simulink model "snap_adc5g_spec"  (R2019a)
settings: Solver=VariableStepDiscrete  StartTime=0.0  StopTime=10.0  RelTol=1e-3
undefined symbols (not defined in the file): pfb_coeff_gen_calc
libraries: xbsIndex_r4 x13965, casper_library_misc x80, casper_library_delays x43, xps_library x5, xbsReplacements_r4 x2, casper_library_communications x1
(part 127 of 152)

== system snap_adc5g_spec/fft_wideband_real/fft_biplex_real_4x/biplex_core/fft_stage_9/butterfly_direct/twiddle/bus_mult ==
  a : Inport
  b : Inport  Port=2
  misci : Inport  Port=3
  a*b_bussify : Subsystem  AncestorBlock=casper_library_flow_control/bus_create  mask(bus_create){inputNum=2}
      mask prompts: inputNum "Number of inputs:"
      mask init:
      | bus_create_init(gcb,...
      |     'inputNum', inputNum);
  a_debus : Subsystem  AncestorBlock=casper_library_flow_control/bus_expand  mask(bus_expand){mode=divisions of arbitrary size, outputNum=1, outputWidth=36, outputBinaryPt=0, outputArithmeticType=0, show_format=on, outputToWorkspace=off, variablePrefix=, outputToModelAsWell=on}
      mask prompts: outputNum "Number of outputs:"; outputWidth "Output width [msb ... lsb]:"; outputBinaryPt "Output binary point position [msb ... lsb]:"; outputArithmeticType "Output arithmetic type (ufix=0, fix=1, bool=2) [msb ... lsb]:"; show_format "Print format string?"; outputToWorkspace "Output to workspace?"; variablePrefix "Variable name prefix:"; outputToModelAsWell "Output to model as well?"
      mask help:
      | Expands a 'bus' made using a bus_create or Xilinx
      | concat block.
      | The input will be divided into the specified number
      | of outputs with the specified arithmetic types.
      | Divisions are made from most significant bit.
      mask init: same as snap_adc5g_spec/ss_adc/ctrl_split
      settings: AttributesFormatString=1 outputs: uf36.0,
      mask TypeOptions mode: divisions of equal size | divisions of arbitrary size
      mask Callback mode: bus_expand_callback();
      mask Callback outputWidth: bus_expand_callback();
      mask Callback outputToWorkspace: bus_expand_callback();
  b_debus : Subsystem  AncestorBlock=casper_library_flow_control/bus_expand  mask(bus_expand){mode=divisions of arbitrary size, outputNum=1, outputWidth=[36 36], outputBinaryPt=[0 0], outputArithmeticType=[0 0], show_format=on, outputToWorkspace=off, variablePrefix=, outputToModelAsWell=on}
      mask prompts: outputNum "Number of outputs:"; outputWidth "Output width [msb ... lsb]:"; outputBinaryPt "Output binary point position [msb ... lsb]:"; outputArithmeticType "Output arithmetic type (ufix=0, fix=1, bool=2) [msb ... lsb]:"; show_format "Print format string?"; outputToWorkspace "Output to workspace?"; variablePrefix "Variable name prefix:"; outputToModelAsWell "Output to model as well?"
      mask help:
      | Expands a 'bus' made using a bus_create or Xilinx
      | concat block.
      | The input will be divided into the specified number
      | of outputs with the specified arithmetic types.
      | Divisions are made from most significant bit.
      mask init: same as snap_adc5g_spec/ss_adc/ctrl_split
      settings: AttributesFormatString=2 outputs: uf36.0,uf36.0,
      mask TypeOptions mode: divisions of equal size | divisions of arbitrary size
      mask Callback mode: bus_expand_callback();
      mask Callback outputWidth: bus_expand_callback();
      mask Callback outputToWorkspace: bus_expand_callback();
  dmisc : xbsIndex_r4/Delay  rst=off  infoeditControl=Selection of Reset will increase slice count due to use of real FFs and instead of SRLs  en=off  latency=mult_latency+add_latency+conv_latency+fan_latency  reg_retiming=on  dbl_ovrd=off  block_type=delay
  mult1 : Subsystem  AncestorBlock=casper_library_multipliers/cmult  mask(cmult){n_bits_a=18, bin_pt_a=17, n_bits_b=18, bin_pt_b=17, n_bits_ab=37, bin_pt_ab=34, quantization=Truncate, overflow=Wrap, conjugated=off, async=off, pipelined_enable=on, floating_point=off, float_type=single, exp_width=8, frac_width=24, in_latency=1, mult_latency=2, add_latency=1, conv_latency=0, pipeline_cmult_en=off, pipeline_latency=0, multiplier_implementation=behavioral HDL}
      mask prompts: n_bits_a "Number of Bits 'a'"; bin_pt_a "Binary Point 'a'"; n_bits_b "Number of Bits 'b'"; bin_pt_b "Binary Point 'b'"; n_bits_ab "Number of Bits 'ab'"; bin_pt_ab "Binary Point 'ab'"; conjugated "Conjugate"; async "asynchronous operation"; pipelined_enable "enable pipeline"; floating_point "floating point"; float_type "float type"; exp_width "exponent width"; frac_width "fraction width"; in_latency "Input latency"; mult_latency "Multiplier Latency"; add_latency "Adder Latency"; conv_latency "Convert latency"; pipeline_cmult_en "Pipeline cmult enable"; pipeline_latency "Pipeline latency"; multiplier_implementation "Multiplier implementation"
      mask help:
      | Multiplies two complex numbers using 4 multipliers and 2 adders.
      | Conjugation is optional.
      mask init: same as snap_adc5g_spec/crosspower_vacc/cmult
      settings: AttributesFormatString=|
      | 18_17 * 18_17 ==> 37_34
      | Truncate, Wrap
      | Latency=1
      mask TypeOptions quantization: Truncate | Round  (unbiased: +/- Inf) | Round  (unbiased: Even Values)
      mask TypeOptions overflow: Wrap | Saturate | Flag as error
      mask Callback floating_point:
      | onoff = get_param(gcb, 'floating_point');
      | if strcmp(onoff,'on')
      |     enable_fixpt = 'off'
      |     set_param_state(gcb, 'float_type', 'on')
      | 
      |     f_type = get_param(gcb, 'float_type')
      |     if strcmp(f_type,'custom')
      |         set_param_state(gcb, 'exp_width', 'on')
      |         set_param_state(gcb, 'frac_width', 'on')
      |     else
      |         set_param_state(gcb, 'exp_width', 'off')
      |         set_param_state(gcb, 'frac_width', 'off')
      |     end
      | 
      | 
      | else
      |     enable_fixpt = 'on'
      |     set_param_state(gcb, 'float_type', 'off')
      |     set_param_state(gcb, 'exp_width', 'off')
      |     set_param_state(gcb, 'frac_width', 'off')
      | end
      | 
      | 
      | set_param_state(gcb, 'n_bits_a', enable_fixpt)
      | set_param_state(gcb, 'bin_pt_a', enable_fixpt)
      | set_param_state(gcb, 'n_bits_b', enable_fixpt)
      | set_param_state(gcb, 'bin_pt_b', enable_fixpt)
      | set_param_state(gcb, 'n_bits_ab', enable_fixpt)
      | set_param_state(gcb, 'bin_pt_ab', enable_fixpt)
      mask TypeOptions float_type: single | custom
      mask Callback float_type:
      | f_type = get_param(gcb, 'float_type')
      | if strcmp(f_type,'custom')
      |     set_param_state(gcb, 'exp_width', 'on')
      |     set_param_state(gcb, 'frac_width', 'on')
      | else
      |     set_param_state(gcb, 'exp_width', 'off')
      |     set_param_state(gcb, 'frac_width', 'off')
      | end
      mask Callback pipeline_cmult_en:
      | pipeline_en = get_param(gcb, 'pipeline_cmult_en');
      | if strcmp(pipeline_en,'on')
      | 
      |     set_param_state(gcb, 'pipeline_latency', 'on')
      | else
      |     set_param_state(gcb, 'pipeline_latency', 'off')
      | end
      mask TypeOptions multiplier_implementation: behavioral HDL | standard core | embedded multiplier core
      mask DialogControl ParameterTabVar0 Prompt: basic
      mask DialogControl ParameterTabVar01 Prompt: latency
      mask DialogControl ParameterTabVar012 Prompt: implementation
  mult2 : Subsystem  AncestorBlock=casper_library_multipliers/cmult  mask(cmult){n_bits_a=18, bin_pt_a=17, n_bits_b=18, bin_pt_b=17, n_bits_ab=37, bin_pt_ab=34, quantization=Truncate, overflow=Wrap, conjugated=off, async=off, pipelined_enable=on, floating_point=off, float_type=single, exp_width=8, frac_width=24, in_latency=1, mult_latency=2, add_latency=1, conv_latency=0, pipeline_cmult_en=off, pipeline_latency=0, multiplier_implementation=behavioral HDL}
      mask prompts: n_bits_a "Number of Bits 'a'"; bin_pt_a "Binary Point 'a'"; n_bits_b "Number of Bits 'b'"; bin_pt_b "Binary Point 'b'"; n_bits_ab "Number of Bits 'ab'"; bin_pt_ab "Binary Point 'ab'"; conjugated "Conjugate"; async "asynchronous operation"; pipelined_enable "enable pipeline"; floating_point "floating point"; float_type "float type"; exp_width "exponent width"; frac_width "fraction width"; in_latency "Input latency"; mult_latency "Multiplier Latency"; add_latency "Adder Latency"; conv_latency "Convert latency"; pipeline_cmult_en "Pipeline cmult enable"; pipeline_latency "Pipeline latency"; multiplier_implementation "Multiplier implementation"
      mask help:
      | Multiplies two complex numbers using 4 multipliers and 2 adders.
      | Conjugation is optional.
      mask init: same as snap_adc5g_spec/crosspower_vacc/cmult
      settings: AttributesFormatString=|
      | 18_17 * 18_17 ==> 37_34
      | Truncate, Wrap
      | Latency=1
      mask TypeOptions quantization: Truncate | Round  (unbiased: +/- Inf) | Round  (unbiased: Even Values)
      mask TypeOptions overflow: Wrap | Saturate | Flag as error
      mask Callback floating_point:
      | onoff = get_param(gcb, 'floating_point');
      | if strcmp(onoff,'on')
      |     enable_fixpt = 'off'
      |     set_param_state(gcb, 'float_type', 'on')
      | 
      |     f_type = get_param(gcb, 'float_type')
      |     if strcmp(f_type,'custom')
      |         set_param_state(gcb, 'exp_width', 'on')
      |         set_param_state(gcb, 'frac_width', 'on')
      |     else
      |         set_param_state(gcb, 'exp_width', 'off')
      |         set_param_state(gcb, 'frac_width', 'off')
      |     end
      | 
      | 
      | else
      |     enable_fixpt = 'on'
      |     set_param_state(gcb, 'float_type', 'off')
      |     set_param_state(gcb, 'exp_width', 'off')
      |     set_param_state(gcb, 'frac_width', 'off')
      | end
      | 
      | 
      | set_param_state(gcb, 'n_bits_a', enable_fixpt)
      | set_param_state(gcb, 'bin_pt_a', enable_fixpt)
      | set_param_state(gcb, 'n_bits_b', enable_fixpt)
      | set_param_state(gcb, 'bin_pt_b', enable_fixpt)
      | set_param_state(gcb, 'n_bits_ab', enable_fixpt)
      | set_param_state(gcb, 'bin_pt_ab', enable_fixpt)
      mask TypeOptions float_type: single | custom
      mask Callback float_type:
      | f_type = get_param(gcb, 'float_type')
      | if strcmp(f_type,'custom')
      |     set_param_state(gcb, 'exp_width', 'on')
      |     set_param_state(gcb, 'frac_width', 'on')
      | else
      |     set_param_state(gcb, 'exp_width', 'off')
      |     set_param_state(gcb, 'frac_width', 'off')
      | end
      mask Callback pipeline_cmult_en:
      | pipeline_en = get_param(gcb, 'pipeline_cmult_en');
      | if strcmp(pipeline_en,'on')
      | 
      |     set_param_state(gcb, 'pipeline_latency', 'on')
      | else
      |     set_param_state(gcb, 'pipeline_latency', 'off')
      | end
      mask TypeOptions multiplier_implementation: behavioral HDL | standard core | embedded multiplier core
      mask DialogControl ParameterTabVar0 Prompt: basic
      mask DialogControl ParameterTabVar01 Prompt: latency
      mask DialogControl ParameterTabVar012 Prompt: implementation
  repa : Subsystem  AncestorBlock=casper_library_bus/bus_replicate  mask(bus_replicate){replication=1, csp_latency=1, misc=off, implementation=core}
      mask prompts: replication "replication factor"; csp_latency "latency"; misc "misc support"; implementation "delay implementation"
      mask help: Output bus formed by replicating input bus a number of times
      mask init:
      | bus_replicate_init(gcb, ...
      |     'replication', replication, ...
      |     'csp_latency', csp_latency, ...
      |     'implementation', implementation, ...
      |     'misc', misc);
      mask TypeOptions implementation: core | behavioral
  repb : Subsystem  AncestorBlock=casper_library_bus/bus_replicate  mask(bus_replicate){replication=1, csp_latency=1, misc=off, implementation=core}
      mask prompts: replication "replication factor"; csp_latency "latency"; misc "misc support"; implementation "delay implementation"
      mask help: Output bus formed by replicating input bus a number of times
      mask init:
      | bus_replicate_init(gcb, ...
      |     'replication', replication, ...
      |     'csp_latency', csp_latency, ...
      |     'implementation', implementation, ...
      |     'misc', misc);
      mask TypeOptions implementation: core | behavioral
  a*b : Outport
  misco : Outport  Port=2
  wires:
  a/1 -> repa/1(in)
  b/1 -> repb/1(in)
  repa/1(out) -> a_debus/1(bus_in)
  repb/1(out) -> b_debus/1(bus_in)
  a_debus/1(msb_lsb_out1) -> mult1/1(a), mult2/1(a)
  b_debus/1(msb_out2) -> mult1/2(b)
  b_debus/2(lsb_out1) -> mult2/2(b)
  misci/1 -> dmisc/1
  mult1/1(ab) -> a*b_bussify/1(in1)
  mult2/1(ab) -> a*b_bussify/2(in2)
  a*b_bussify/1(bus_out) -> a*b/1
  dmisc/1 -> misco/1

== system snap_adc5g_spec/fft_wideband_real/fft_biplex_real_4x/biplex_core/fft_stage_9/butterfly_direct/twiddle/coeff_gen ==
  rst : Inport
  misci : Inport  Port=2
  Counter : xbsIndex_r4/Counter  cnt_type=Free Running  cnt_to=Inf  operation=Up  start_count=0  cnt_by_val=1  arith_type=Unsigned  n_bits=10  bin_pt=0  load_pin=off  rst=on  en=off  explicit_period=on  period=1  use_behavioral_HDL=on  implementation=Fabric  dbl_ovrd=off  block_type=counter
  Slice : xbsIndex_r4/Slice  nbits=8  boolean_output=off  mode=Upper Bit Location + Width  bit1=0  base1=MSB of Input  bit0=0  base0=LSB of Input  dbl_ovrd=off  block_type=slice
  bit_reverse : Subsystem  AncestorBlock=casper_library_misc/bit_reverse  mask(bit_reverse){n_bits=8}
      mask prompts: n_bits "Number of Bits"
      mask help: Reverses the bit order of the input. Input must be unsigned with binary point at position 0. Costs nothing in hardware.
      mask init:
      | bit_reverse_init(gcb,'n_bits', n_bits);
      settings: AttributesFormatString=8 bits
      mask Help: eval('xlWeb(''http://casper.berkeley.edu/wiki/Bit_reverse'')')
  cosin : Subsystem  Tag=casper:cosin  AncestorBlock=casper_library_downconverter/cosin  mask(cosin){output0=cos, output1=-sin, indep_theta=off, phase=0, fraction=1, table_bits=8, n_bits=18, bin_pt=17, floating_point=off, float_type=single, exp_width=8, frac_width=24, store=1, pack=on, bram=BRAM, misc=on, bram_latency=3, add_latency=1, mux_latency=2, neg_latency=2, conv_latency=1}
      mask prompts: output0 "first output function"; output1 "second output function"; indep_theta "Independent theta values"; phase "initial phase offset (?*(2*pi))"; fraction "fraction of cycle period to output (1/2^?)"; table_bits "samples in cycle period fraction to output (2^?)"; n_bits "bit width"; bin_pt "binary point"; floating_point "floating point"; float_type "float type"; exp_width "exponent width"; frac_width "fraction width"; store "fraction of cycle period to store (1/2^?)"; pack "pack lookup values in same output word"; bram "BRAM implementation"; misc "Miscellaneous port"; bram_latency "bram latency"; add_latency "large adder latency"; mux_latency "mux latency"; neg_latency "negate latency"; conv_latency "convert latency"
      mask init: same as snap_adc5g_spec/fft_wideband_real/fft_direct/butterfly0_0/twiddle/coeff_gen/cosin
      mask TypeOptions output0: sin | cos | -sin | -cos
      mask TypeOptions output1: none | sin | cos | -sin | -cos
      mask Callback floating_point:
      | onoff = get_param(gcb, 'floating_point');
      | if strcmp(onoff,'on')
      |     enable_fixpt = 'off';
      |     set_param_state(gcb, 'float_type', 'on')
      | 
      |     f_type = get_param(gcb, 'float_type');
      |     if strcmp(f_type,'custom')
      |         set_param_state(gcb, 'exp_width', 'on')
      |         set_param_state(gcb, 'frac_width', 'on')
      |     else
      |         set_param_state(gcb, 'exp_width', 'off')
      |         set_param_state(gcb, 'frac_width', 'off')
      |     end
      | 
      | 
      | else
      |     enable_fixpt = 'on';
      |     set_param_state(gcb, 'float_type', 'off')
      |     set_param_state(gcb, 'exp_width', 'off')
      |     set_param_state(gcb, 'frac_width', 'off')
      | end
      | 
      | set_param_state(gcb, 'n_bits', enable_fixpt)
      | set_param_state(gcb, 'bin_pt', enable_fixpt)
      mask TypeOptions float_type: single | custom
      mask Callback float_type:
      | f_type = get_param(gcb, 'float_type');
      | if strcmp(f_type,'custom')
      |     set_param_state(gcb, 'exp_width', 'on')
      |     set_param_state(gcb, 'frac_width', 'on')
      | else
      |     set_param_state(gcb, 'exp_width', 'off')
      |     set_param_state(gcb, 'frac_width', 'off')
      | end
      mask TypeOptions bram: distributed RAM | BRAM
      mask Display:
      | if ~(table_bits == 0),
      |         color('black');port_label('output',1,output0);
      |     color('black');port_label('output',2,output1);
      |     color('black');disp(['z^{-',num2str(add_latency+mux_latency+conv_latency+bram_latency+neg_latency+mux_latency),'}'],'texmode','on');color('black');port_label('input',1,'theta');
      |     if strcmp(misc, 'on'),
      |         color('black');port_label('input',2,'misci');
      |         color('black');port_label('output',3,'misco');
      |     end
      | end
  ri_to_c : casper_library_misc/ri_to_c
      settings: SourceProductName=CASPER DSP Blockset
  w : Outport
  misco : Outport  Port=2
  wires:
  ri_to_c/1 -> w/1
  rst/1 -> Counter/1
  Counter/1 -> Slice/1
  Slice/1 -> bit_reverse/1(in)
  bit_reverse/1(out) -> cosin/1(theta)
  cosin/1(cos) -> ri_to_c/1
  cosin/2(-sin) -> ri_to_c/2
  misci/1 -> cosin/2(misci)
  cosin/3(misco) -> misco/1

== system snap_adc5g_spec/fft_wideband_real/fft_direct/butterfly0_0/twiddle/bus_mult/mult1/a_expand ==
  bus_in : Inport
  reinterpret{1..4} (4 alike) : xbsIndex_r4/Reinterpret  force_arith_type=on  arith_type="Signed  (2's comp)"  force_bin_pt=on  bin_pt=17  block_type=reinterpret
  slice1 : xbsIndex_r4/Slice  nbits=18  boolean_output=off  mode=Upper Bit Location + Width  bit1=-54  base1=MSB of Input  bit0=0  base0=LSB of Input  dbl_ovrd=off  block_type=slice
  slice2 : xbsIndex_r4/Slice  nbits=18  boolean_output=off  mode=Upper Bit Location + Width  bit1=-36  base1=MSB of Input  bit0=0  base0=LSB of Input  dbl_ovrd=off  block_type=slice
  slice3 : xbsIndex_r4/Slice  nbits=18  boolean_output=off  mode=Upper Bit Location + Width  bit1=-18  base1=MSB of Input  bit0=0  base0=LSB of Input  dbl_ovrd=off  block_type=slice
  slice4 : xbsIndex_r4/Slice  nbits=18  boolean_output=off  mode=Upper Bit Location + Width  bit1=0  base1=MSB of Input  bit0=0  base0=LSB of Input  dbl_ovrd=off  block_type=slice
  msb_out4 : Outport
  out3 : Outport  Port=2
  out2 : Outport  Port=3
  lsb_out1 : Outport  Port=4
  wires:
  bus_in/1 -> slice4/1, slice3/1, slice2/1, slice1/1
  slice4/1 -> reinterpret4/1
  reinterpret4/1 -> msb_out4/1
  slice3/1 -> reinterpret3/1
  reinterpret3/1 -> out3/1
  slice2/1 -> reinterpret2/1
  reinterpret2/1 -> out2/1
  slice1/1 -> reinterpret1/1
  reinterpret1/1 -> lsb_out1/1

== system snap_adc5g_spec/fft_wideband_real/fft_direct/butterfly0_0/twiddle/bus_mult/mult1/a_replicate ==
  in : Inport
  bussify : Subsystem  AncestorBlock=casper_library_flow_control/bus_create  mask(bus_create){inputNum=2}
      mask prompts: inputNum "Number of inputs:"
      mask init:
      | bus_create_init(gcb,...
      |     'inputNum', inputNum);
  din0_0 : xbsIndex_r4/Delay  rst=off  infoeditControl=Selection of Reset will increase slice count due to use of real FFs and instead of SRLs  en=off  latency=1  reg_retiming=off  dbl_ovrd=off  block_type=delay
  din0_1 : xbsIndex_r4/Delay  rst=off  infoeditControl=Selection of Reset will increase slice count due to use of real FFs and instead of SRLs  en=off  latency=1  reg_retiming=off  dbl_ovrd=off  block_type=delay
  out : Outport
  wires:
  in/1 -> din0_0/1, din0_1/1
  din0_0/1 -> bussify/1(in1)
  din0_1/1 -> bussify/2(in2)
  bussify/1(bus_out) -> out/1

== system snap_adc5g_spec/fft_wideband_real/fft_direct/butterfly0_0/twiddle/bus_mult/mult1/b_expand ==
  bus_in : Inport
  reinterpret{1..4} (4 alike) : xbsIndex_r4/Reinterpret  force_arith_type=on  arith_type="Signed  (2's comp)"  force_bin_pt=on  bin_pt=17  block_type=reinterpret
  slice1 : xbsIndex_r4/Slice  nbits=18  boolean_output=off  mode=Upper Bit Location + Width  bit1=-54  base1=MSB of Input  bit0=0  base0=LSB of Input  dbl_ovrd=off  block_type=slice
  slice2 : xbsIndex_r4/Slice  nbits=18  boolean_output=off  mode=Upper Bit Location + Width  bit1=-36  base1=MSB of Input  bit0=0  base0=LSB of Input  dbl_ovrd=off  block_type=slice
  slice3 : xbsIndex_r4/Slice  nbits=18  boolean_output=off  mode=Upper Bit Location + Width  bit1=-18  base1=MSB of Input  bit0=0  base0=LSB of Input  dbl_ovrd=off  block_type=slice
  slice4 : xbsIndex_r4/Slice  nbits=18  boolean_output=off  mode=Upper Bit Location + Width  bit1=0  base1=MSB of Input  bit0=0  base0=LSB of Input  dbl_ovrd=off  block_type=slice
  msb_out4 : Outport
  out3 : Outport  Port=2
  out2 : Outport  Port=3
  lsb_out1 : Outport  Port=4
  wires:
  bus_in/1 -> slice4/1, slice3/1, slice2/1, slice1/1
  slice4/1 -> reinterpret4/1
  reinterpret4/1 -> msb_out4/1
  slice3/1 -> reinterpret3/1
  reinterpret3/1 -> out3/1
  slice2/1 -> reinterpret2/1
  reinterpret2/1 -> out2/1
  slice1/1 -> reinterpret1/1
  reinterpret1/1 -> lsb_out1/1

== system snap_adc5g_spec/fft_wideband_real/fft_direct/butterfly0_0/twiddle/bus_mult/mult1/b_replicate ==
  in : Inport
  bussify : Subsystem  AncestorBlock=casper_library_flow_control/bus_create  mask(bus_create){inputNum=2}
      mask prompts: inputNum "Number of inputs:"
      mask init:
      | bus_create_init(gcb,...
      |     'inputNum', inputNum);
  din0_0 : xbsIndex_r4/Delay  rst=off  infoeditControl=Selection of Reset will increase slice count due to use of real FFs and instead of SRLs  en=off  latency=1  reg_retiming=off  dbl_ovrd=off  block_type=delay
  din0_1 : xbsIndex_r4/Delay  rst=off  infoeditControl=Selection of Reset will increase slice count due to use of real FFs and instead of SRLs  en=off  latency=1  reg_retiming=off  dbl_ovrd=off  block_type=delay
  out : Outport
  wires:
  in/1 -> din0_0/1, din0_1/1
  din0_0/1 -> bussify/1(in1)
  din0_1/1 -> bussify/2(in2)
  bussify/1(bus_out) -> out/1

== system snap_adc5g_spec/fft_wideband_real/fft_direct/butterfly0_0/twiddle/bus_mult/mult1/ri_to_c ==
  re : Inport
  im : Inport  Port=2
  concat : xbsIndex_r4/Concat  num_inputs=2  dbl_ovrd=off  block_type=concat
      settings: block_version=9.1.01
  force_im : xbsIndex_r4/Reinterpret  force_arith_type=on  arith_type=Unsigned  force_bin_pt=on  bin_pt=0  block_type=reinterpret
      settings: infoedit="Changes signal type without altering the binary representation.   You can changed the signal between signed and unsigned, and relocate the binary point.<P><P>Hardware notes: In hardware this block costs nothing.<P><P>Example:  Suppose the input is 6 bits wide, signed, with 2 fractional bits, and the output is forced to unsigned with 0 fractional bits.  Then an input of -2.0 (1110.00 in binary 2's complement) becomes an output of 56 (111000 in binary)."  block_version=9.1.01
  force_re : xbsIndex_r4/Reinterpret  force_arith_type=on  arith_type=Unsigned  force_bin_pt=on  bin_pt=0  block_type=reinterpret
      settings: infoedit="Changes signal type without altering the binary representation.   You can changed the signal between signed and unsigned, and relocate the binary point.<P><P>Hardware notes: In hardware this block costs nothing.<P><P>Example:  Suppose the input is 6 bits wide, signed, with 2 fractional bits, and the output is forced to unsigned with 0 fractional bits.  Then an input of -2.0 (1110.00 in binary 2's complement) becomes an output of 56 (111000 in binary)."  block_version=9.1.01
  c : Outport
  wires:
  force_re/1 -> concat/1
  force_im/1 -> concat/2
  re/1 -> force_re/1
  concat/1 -> c/1
  im/1 -> force_im/1

== system snap_adc5g_spec/fft_wideband_real/fft_direct/butterfly0_0/twiddle/bus_mult/mult2/a_expand ==
  bus_in : Inport
  reinterpret{1..4} (4 alike) : xbsIndex_r4/Reinterpret  force_arith_type=on  arith_type="Signed  (2's comp)"  force_bin_pt=on  bin_pt=17  block_type=reinterpret
  slice1 : xbsIndex_r4/Slice  nbits=18  boolean_output=off  mode=Upper Bit Location + Width  bit1=-54  base1=MSB of Input  bit0=0  base0=LSB of Input  dbl_ovrd=off  block_type=slice
  slice2 : xbsIndex_r4/Slice  nbits=18  boolean_output=off  mode=Upper Bit Location + Width  bit1=-36  base1=MSB of Input  bit0=0  base0=LSB of Input  dbl_ovrd=off  block_type=slice
  slice3 : xbsIndex_r4/Slice  nbits=18  boolean_output=off  mode=Upper Bit Location + Width  bit1=-18  base1=MSB of Input  bit0=0  base0=LSB of Input  dbl_ovrd=off  block_type=slice
  slice4 : xbsIndex_r4/Slice  nbits=18  boolean_output=off  mode=Upper Bit Location + Width  bit1=0  base1=MSB of Input  bit0=0  base0=LSB of Input  dbl_ovrd=off  block_type=slice
  msb_out4 : Outport
  out3 : Outport  Port=2
  out2 : Outport  Port=3
  lsb_out1 : Outport  Port=4
  wires:
  bus_in/1 -> slice4/1, slice3/1, slice2/1, slice1/1
  slice4/1 -> reinterpret4/1
  reinterpret4/1 -> msb_out4/1
  slice3/1 -> reinterpret3/1
  reinterpret3/1 -> out3/1
  slice2/1 -> reinterpret2/1
  reinterpret2/1 -> out2/1
  slice1/1 -> reinterpret1/1
  reinterpret1/1 -> lsb_out1/1

== system snap_adc5g_spec/fft_wideband_real/fft_direct/butterfly0_0/twiddle/bus_mult/mult2/a_replicate ==
  in : Inport
  bussify : Subsystem  AncestorBlock=casper_library_flow_control/bus_create  mask(bus_create){inputNum=2}
      mask prompts: inputNum "Number of inputs:"
      mask init:
      | bus_create_init(gcb,...
      |     'inputNum', inputNum);
  din0_0 : xbsIndex_r4/Delay  rst=off  infoeditControl=Selection of Reset will increase slice count due to use of real FFs and instead of SRLs  en=off  latency=1  reg_retiming=off  dbl_ovrd=off  block_type=delay
  din0_1 : xbsIndex_r4/Delay  rst=off  infoeditControl=Selection of Reset will increase slice count due to use of real FFs and instead of SRLs  en=off  latency=1  reg_retiming=off  dbl_ovrd=off  block_type=delay
  out : Outport
  wires:
  in/1 -> din0_0/1, din0_1/1
  din0_0/1 -> bussify/1(in1)
  din0_1/1 -> bussify/2(in2)
  bussify/1(bus_out) -> out/1

== system snap_adc5g_spec/fft_wideband_real/fft_direct/butterfly0_0/twiddle/bus_mult/mult2/b_expand ==
  bus_in : Inport
  reinterpret{1..4} (4 alike) : xbsIndex_r4/Reinterpret  force_arith_type=on  arith_type="Signed  (2's comp)"  force_bin_pt=on  bin_pt=17  block_type=reinterpret
  slice1 : xbsIndex_r4/Slice  nbits=18  boolean_output=off  mode=Upper Bit Location + Width  bit1=-54  base1=MSB of Input  bit0=0  base0=LSB of Input  dbl_ovrd=off  block_type=slice
  slice2 : xbsIndex_r4/Slice  nbits=18  boolean_output=off  mode=Upper Bit Location + Width  bit1=-36  base1=MSB of Input  bit0=0  base0=LSB of Input  dbl_ovrd=off  block_type=slice
  slice3 : xbsIndex_r4/Slice  nbits=18  boolean_output=off  mode=Upper Bit Location + Width  bit1=-18  base1=MSB of Input  bit0=0  base0=LSB of Input  dbl_ovrd=off  block_type=slice
  slice4 : xbsIndex_r4/Slice  nbits=18  boolean_output=off  mode=Upper Bit Location + Width  bit1=0  base1=MSB of Input  bit0=0  base0=LSB of Input  dbl_ovrd=off  block_type=slice
  msb_out4 : Outport
  out3 : Outport  Port=2
  out2 : Outport  Port=3
  lsb_out1 : Outport  Port=4
  wires:
  bus_in/1 -> slice4/1, slice3/1, slice2/1, slice1/1
  slice4/1 -> reinterpret4/1
  reinterpret4/1 -> msb_out4/1
  slice3/1 -> reinterpret3/1
  reinterpret3/1 -> out3/1
  slice2/1 -> reinterpret2/1
  reinterpret2/1 -> out2/1
  slice1/1 -> reinterpret1/1
  reinterpret1/1 -> lsb_out1/1

== system snap_adc5g_spec/fft_wideband_real/fft_direct/butterfly0_0/twiddle/bus_mult/mult2/b_replicate ==
  in : Inport
  bussify : Subsystem  AncestorBlock=casper_library_flow_control/bus_create  mask(bus_create){inputNum=2}
      mask prompts: inputNum "Number of inputs:"
      mask init:
      | bus_create_init(gcb,...
      |     'inputNum', inputNum);
  din0_0 : xbsIndex_r4/Delay  rst=off  infoeditControl=Selection of Reset will increase slice count due to use of real FFs and instead of SRLs  en=off  latency=1  reg_retiming=off  dbl_ovrd=off  block_type=delay
  din0_1 : xbsIndex_r4/Delay  rst=off  infoeditControl=Selection of Reset will increase slice count due to use of real FFs and instead of SRLs  en=off  latency=1  reg_retiming=off  dbl_ovrd=off  block_type=delay
  out : Outport
  wires:
  in/1 -> din0_0/1, din0_1/1
  din0_0/1 -> bussify/1(in1)
  din0_1/1 -> bussify/2(in2)
  bussify/1(bus_out) -> out/1

== system snap_adc5g_spec/fft_wideband_real/fft_direct/butterfly0_0/twiddle/bus_mult/mult2/ri_to_c ==
  re : Inport
  im : Inport  Port=2
  concat : xbsIndex_r4/Concat  num_inputs=2  dbl_ovrd=off  block_type=concat
      settings: block_version=9.1.01
  force_im : xbsIndex_r4/Reinterpret  force_arith_type=on  arith_type=Unsigned  force_bin_pt=on  bin_pt=0  block_type=reinterpret
      settings: infoedit="Changes signal type without altering the binary representation.   You can changed the signal between signed and unsigned, and relocate the binary point.<P><P>Hardware notes: In hardware this block costs nothing.<P><P>Example:  Suppose the input is 6 bits wide, signed, with 2 fractional bits, and the output is forced to unsigned with 0 fractional bits.  Then an input of -2.0 (1110.00 in binary 2's complement) becomes an output of 56 (111000 in binary)."  block_version=9.1.01
  force_re : xbsIndex_r4/Reinterpret  force_arith_type=on  arith_type=Unsigned  force_bin_pt=on  bin_pt=0  block_type=reinterpret
      settings: infoedit="Changes signal type without altering the binary representation.   You can changed the signal between signed and unsigned, and relocate the binary point.<P><P>Hardware notes: In hardware this block costs nothing.<P><P>Example:  Suppose the input is 6 bits wide, signed, with 2 fractional bits, and the output is forced to unsigned with 0 fractional bits.  Then an input of -2.0 (1110.00 in binary 2's complement) becomes an output of 56 (111000 in binary)."  block_version=9.1.01
  c : Outport
  wires:
  force_re/1 -> concat/1
  force_im/1 -> concat/2
  re/1 -> force_re/1
  concat/1 -> c/1
  im/1 -> force_im/1

== system snap_adc5g_spec/fft_wideband_real/fft_direct/butterfly0_0/twiddle/bus_mult/mult3/a_expand ==
  bus_in : Inport
  reinterpret{1..4} (4 alike) : xbsIndex_r4/Reinterpret  force_arith_type=on  arith_type="Signed  (2's comp)"  force_bin_pt=on  bin_pt=17  block_type=reinterpret
  slice1 : xbsIndex_r4/Slice  nbits=18  boolean_output=off  mode=Upper Bit Location + Width  bit1=-54  base1=MSB of Input  bit0=0  base0=LSB of Input  dbl_ovrd=off  block_type=slice
  slice2 : xbsIndex_r4/Slice  nbits=18  boolean_output=off  mode=Upper Bit Location + Width  bit1=-36  base1=MSB of Input  bit0=0  base0=LSB of Input  dbl_ovrd=off  block_type=slice
  slice3 : xbsIndex_r4/Slice  nbits=18  boolean_output=off  mode=Upper Bit Location + Width  bit1=-18  base1=MSB of Input  bit0=0  base0=LSB of Input  dbl_ovrd=off  block_type=slice
  slice4 : xbsIndex_r4/Slice  nbits=18  boolean_output=off  mode=Upper Bit Location + Width  bit1=0  base1=MSB of Input  bit0=0  base0=LSB of Input  dbl_ovrd=off  block_type=slice
  msb_out4 : Outport
  out3 : Outport  Port=2
  out2 : Outport  Port=3
  lsb_out1 : Outport  Port=4
  wires:
  bus_in/1 -> slice4/1, slice3/1, slice2/1, slice1/1
  slice4/1 -> reinterpret4/1
  reinterpret4/1 -> msb_out4/1
  slice3/1 -> reinterpret3/1
  reinterpret3/1 -> out3/1
  slice2/1 -> reinterpret2/1
  reinterpret2/1 -> out2/1
  slice1/1 -> reinterpret1/1
  reinterpret1/1 -> lsb_out1/1

== system snap_adc5g_spec/fft_wideband_real/fft_direct/butterfly0_0/twiddle/bus_mult/mult3/a_replicate ==
  in : Inport
  bussify : Subsystem  AncestorBlock=casper_library_flow_control/bus_create  mask(bus_create){inputNum=2}
      mask prompts: inputNum "Number of inputs:"
      mask init:
      | bus_create_init(gcb,...
      |     'inputNum', inputNum);
  din0_0 : xbsIndex_r4/Delay  rst=off  infoeditControl=Selection of Reset will increase slice count due to use of real FFs and instead of SRLs  en=off  latency=1  reg_retiming=off  dbl_ovrd=off  block_type=delay
  din0_1 : xbsIndex_r4/Delay  rst=off  infoeditControl=Selection of Reset will increase slice count due to use of real FFs and instead of SRLs  en=off  latency=1  reg_retiming=off  dbl_ovrd=off  block_type=delay
  out : Outport
  wires:
  in/1 -> din0_0/1, din0_1/1
  din0_0/1 -> bussify/1(in1)
  din0_1/1 -> bussify/2(in2)
  bussify/1(bus_out) -> out/1

== system snap_adc5g_spec/fft_wideband_real/fft_direct/butterfly0_0/twiddle/bus_mult/mult3/b_expand ==
  bus_in : Inport
  reinterpret{1..4} (4 alike) : xbsIndex_r4/Reinterpret  force_arith_type=on  arith_type="Signed  (2's comp)"  force_bin_pt=on  bin_pt=17  block_type=reinterpret
  slice1 : xbsIndex_r4/Slice  nbits=18  boolean_output=off  mode=Upper Bit Location + Width  bit1=-54  base1=MSB of Input  bit0=0  base0=LSB of Input  dbl_ovrd=off  block_type=slice
  slice2 : xbsIndex_r4/Slice  nbits=18  boolean_output=off  mode=Upper Bit Location + Width  bit1=-36  base1=MSB of Input  bit0=0  base0=LSB of Input  dbl_ovrd=off  block_type=slice
  slice3 : xbsIndex_r4/Slice  nbits=18  boolean_output=off  mode=Upper Bit Location + Width  bit1=-18  base1=MSB of Input  bit0=0  base0=LSB of Input  dbl_ovrd=off  block_type=slice
  slice4 : xbsIndex_r4/Slice  nbits=18  boolean_output=off  mode=Upper Bit Location + Width  bit1=0  base1=MSB of Input  bit0=0  base0=LSB of Input  dbl_ovrd=off  block_type=slice
  msb_out4 : Outport
  out3 : Outport  Port=2
  out2 : Outport  Port=3
  lsb_out1 : Outport  Port=4
  wires:
  bus_in/1 -> slice4/1, slice3/1, slice2/1, slice1/1
  slice4/1 -> reinterpret4/1
  reinterpret4/1 -> msb_out4/1
  slice3/1 -> reinterpret3/1
  reinterpret3/1 -> out3/1
  slice2/1 -> reinterpret2/1
  reinterpret2/1 -> out2/1
  slice1/1 -> reinterpret1/1
  reinterpret1/1 -> lsb_out1/1

== system snap_adc5g_spec/fft_wideband_real/fft_direct/butterfly0_0/twiddle/bus_mult/mult3/b_replicate ==
  in : Inport
  bussify : Subsystem  AncestorBlock=casper_library_flow_control/bus_create  mask(bus_create){inputNum=2}
      mask prompts: inputNum "Number of inputs:"
      mask init:
      | bus_create_init(gcb,...
      |     'inputNum', inputNum);
  din0_0 : xbsIndex_r4/Delay  rst=off  infoeditControl=Selection of Reset will increase slice count due to use of real FFs and instead of SRLs  en=off  latency=1  reg_retiming=off  dbl_ovrd=off  block_type=delay
  din0_1 : xbsIndex_r4/Delay  rst=off  infoeditControl=Selection of Reset will increase slice count due to use of real FFs and instead of SRLs  en=off  latency=1  reg_retiming=off  dbl_ovrd=off  block_type=delay
  out : Outport
  wires:
  in/1 -> din0_0/1, din0_1/1
  din0_0/1 -> bussify/1(in1)
  din0_1/1 -> bussify/2(in2)
  bussify/1(bus_out) -> out/1

== system snap_adc5g_spec/fft_wideband_real/fft_direct/butterfly0_0/twiddle/bus_mult/mult3/ri_to_c ==
  re : Inport
  im : Inport  Port=2
  concat : xbsIndex_r4/Concat  num_inputs=2  dbl_ovrd=off  block_type=concat
      settings: block_version=9.1.01
  force_im : xbsIndex_r4/Reinterpret  force_arith_type=on  arith_type=Unsigned  force_bin_pt=on  bin_pt=0  block_type=reinterpret
      settings: infoedit="Changes signal type without altering the binary representation.   You can changed the signal between signed and unsigned, and relocate the binary point.<P><P>Hardware notes: In hardware this block costs nothing.<P><P>Example:  Suppose the input is 6 bits wide, signed, with 2 fractional bits, and the output is forced to unsigned with 0 fractional bits.  Then an input of -2.0 (1110.00 in binary 2's complement) becomes an output of 56 (111000 in binary)."  block_version=9.1.01
  force_re : xbsIndex_r4/Reinterpret  force_arith_type=on  arith_type=Unsigned  force_bin_pt=on  bin_pt=0  block_type=reinterpret
      settings: infoedit="Changes signal type without altering the binary representation.   You can changed the signal between signed and unsigned, and relocate the binary point.<P><P>Hardware notes: In hardware this block costs nothing.<P><P>Example:  Suppose the input is 6 bits wide, signed, with 2 fractional bits, and the output is forced to unsigned with 0 fractional bits.  Then an input of -2.0 (1110.00 in binary 2's complement) becomes an output of 56 (111000 in binary)."  block_version=9.1.01
  c : Outport
  wires:
  force_re/1 -> concat/1
  force_im/1 -> concat/2
  re/1 -> force_re/1
  concat/1 -> c/1
  im/1 -> force_im/1

== system snap_adc5g_spec/fft_wideband_real/fft_direct/butterfly0_0/twiddle/bus_mult/mult4/a_expand ==
  bus_in : Inport
  reinterpret{1..4} (4 alike) : xbsIndex_r4/Reinterpret  force_arith_type=on  arith_type="Signed  (2's comp)"  force_bin_pt=on  bin_pt=17  block_type=reinterpret
  slice1 : xbsIndex_r4/Slice  nbits=18  boolean_output=off  mode=Upper Bit Location + Width  bit1=-54  base1=MSB of Input  bit0=0  base0=LSB of Input  dbl_ovrd=off  block_type=slice
  slice2 : xbsIndex_r4/Slice  nbits=18  boolean_output=off  mode=Upper Bit Location + Width  bit1=-36  base1=MSB of Input  bit0=0  base0=LSB of Input  dbl_ovrd=off  block_type=slice
  slice3 : xbsIndex_r4/Slice  nbits=18  boolean_output=off  mode=Upper Bit Location + Width  bit1=-18  base1=MSB of Input  bit0=0  base0=LSB of Input  dbl_ovrd=off  block_type=slice
  slice4 : xbsIndex_r4/Slice  nbits=18  boolean_output=off  mode=Upper Bit Location + Width  bit1=0  base1=MSB of Input  bit0=0  base0=LSB of Input  dbl_ovrd=off  block_type=slice
  msb_out4 : Outport
  out3 : Outport  Port=2
  out2 : Outport  Port=3
  lsb_out1 : Outport  Port=4
  wires:
  bus_in/1 -> slice4/1, slice3/1, slice2/1, slice1/1
  slice4/1 -> reinterpret4/1
  reinterpret4/1 -> msb_out4/1
  slice3/1 -> reinterpret3/1
  reinterpret3/1 -> out3/1
  slice2/1 -> reinterpret2/1
  reinterpret2/1 -> out2/1
  slice1/1 -> reinterpret1/1
  reinterpret1/1 -> lsb_out1/1

== system snap_adc5g_spec/fft_wideband_real/fft_direct/butterfly0_0/twiddle/bus_mult/mult4/a_replicate ==
  in : Inport
  bussify : Subsystem  AncestorBlock=casper_library_flow_control/bus_create  mask(bus_create){inputNum=2}
      mask prompts: inputNum "Number of inputs:"
      mask init:
      | bus_create_init(gcb,...
      |     'inputNum', inputNum);
  din0_0 : xbsIndex_r4/Delay  rst=off  infoeditControl=Selection of Reset will increase slice count due to use of real FFs and instead of SRLs  en=off  latency=1  reg_retiming=off  dbl_ovrd=off  block_type=delay
  din0_1 : xbsIndex_r4/Delay  rst=off  infoeditControl=Selection of Reset will increase slice count due to use of real FFs and instead of SRLs  en=off  latency=1  reg_retiming=off  dbl_ovrd=off  block_type=delay
  out : Outport
  wires:
  in/1 -> din0_0/1, din0_1/1
  din0_0/1 -> bussify/1(in1)
  din0_1/1 -> bussify/2(in2)
  bussify/1(bus_out) -> out/1

== system snap_adc5g_spec/fft_wideband_real/fft_direct/butterfly0_0/twiddle/bus_mult/mult4/b_expand ==
  bus_in : Inport
  reinterpret{1..4} (4 alike) : xbsIndex_r4/Reinterpret  force_arith_type=on  arith_type="Signed  (2's comp)"  force_bin_pt=on  bin_pt=17  block_type=reinterpret
  slice1 : xbsIndex_r4/Slice  nbits=18  boolean_output=off  mode=Upper Bit Location + Width  bit1=-54  base1=MSB of Input  bit0=0  base0=LSB of Input  dbl_ovrd=off  block_type=slice
  slice2 : xbsIndex_r4/Slice  nbits=18  boolean_output=off  mode=Upper Bit Location + Width  bit1=-36  base1=MSB of Input  bit0=0  base0=LSB of Input  dbl_ovrd=off  block_type=slice
  slice3 : xbsIndex_r4/Slice  nbits=18  boolean_output=off  mode=Upper Bit Location + Width  bit1=-18  base1=MSB of Input  bit0=0  base0=LSB of Input  dbl_ovrd=off  block_type=slice
  slice4 : xbsIndex_r4/Slice  nbits=18  boolean_output=off  mode=Upper Bit Location + Width  bit1=0  base1=MSB of Input  bit0=0  base0=LSB of Input  dbl_ovrd=off  block_type=slice
  msb_out4 : Outport
  out3 : Outport  Port=2
  out2 : Outport  Port=3
  lsb_out1 : Outport  Port=4
  wires:
  bus_in/1 -> slice4/1, slice3/1, slice2/1, slice1/1
  slice4/1 -> reinterpret4/1
  reinterpret4/1 -> msb_out4/1
  slice3/1 -> reinterpret3/1
  reinterpret3/1 -> out3/1
  slice2/1 -> reinterpret2/1
  reinterpret2/1 -> out2/1
  slice1/1 -> reinterpret1/1
  reinterpret1/1 -> lsb_out1/1

== system snap_adc5g_spec/fft_wideband_real/fft_direct/butterfly0_0/twiddle/bus_mult/mult4/b_replicate ==
  in : Inport
  bussify : Subsystem  AncestorBlock=casper_library_flow_control/bus_create  mask(bus_create){inputNum=2}
      mask prompts: inputNum "Number of inputs:"
      mask init:
      | bus_create_init(gcb,...
      |     'inputNum', inputNum);
  din0_0 : xbsIndex_r4/Delay  rst=off  infoeditControl=Selection of Reset will increase slice count due to use of real FFs and instead of SRLs  en=off  latency=1  reg_retiming=off  dbl_ovrd=off  block_type=delay
  din0_1 : xbsIndex_r4/Delay  rst=off  infoeditControl=Selection of Reset will increase slice count due to use of real FFs and instead of SRLs  en=off  latency=1  reg_retiming=off  dbl_ovrd=off  block_type=delay
  out : Outport
  wires:
  in/1 -> din0_0/1, din0_1/1
  din0_0/1 -> bussify/1(in1)
  din0_1/1 -> bussify/2(in2)
  bussify/1(bus_out) -> out/1

== system snap_adc5g_spec/fft_wideband_real/fft_direct/butterfly0_0/twiddle/bus_mult/mult4/ri_to_c ==
  re : Inport
  im : Inport  Port=2
  concat : xbsIndex_r4/Concat  num_inputs=2  dbl_ovrd=off  block_type=concat
      settings: block_version=9.1.01
  force_im : xbsIndex_r4/Reinterpret  force_arith_type=on  arith_type=Unsigned  force_bin_pt=on  bin_pt=0  block_type=reinterpret
      settings: infoedit="Changes signal type without altering the binary representation.   You can changed the signal between signed and unsigned, and relocate the binary point.<P><P>Hardware notes: In hardware this block costs nothing.<P><P>Example:  Suppose the input is 6 bits wide, signed, with 2 fractional bits, and the output is forced to unsigned with 0 fractional bits.  Then an input of -2.0 (1110.00 in binary 2's complement) becomes an output of 56 (111000 in binary)."  block_version=9.1.01
  force_re : xbsIndex_r4/Reinterpret  force_arith_type=on  arith_type=Unsigned  force_bin_pt=on  bin_pt=0  block_type=reinterpret
      settings: infoedit="Changes signal type without altering the binary representation.   You can changed the signal between signed and unsigned, and relocate the binary point.<P><P>Hardware notes: In hardware this block costs nothing.<P><P>Example:  Suppose the input is 6 bits wide, signed, with 2 fractional bits, and the output is forced to unsigned with 0 fractional bits.  Then an input of -2.0 (1110.00 in binary 2's complement) becomes an output of 56 (111000 in binary)."  block_version=9.1.01
  c : Outport
  wires:
  force_re/1 -> concat/1
  force_im/1 -> concat/2
  re/1 -> force_re/1
  concat/1 -> c/1
  im/1 -> force_im/1

== system snap_adc5g_spec/fft_wideband_real/fft_direct/butterfly0_0/twiddle/bus_mult/repa/bussify ==
  in1 : Inport
  reinterpret1 : xbsIndex_r4/Reinterpret  force_arith_type=on  arith_type=Unsigned  force_bin_pt=on  bin_pt=0  block_type=reinterpret
      settings: infoedit="Changes signal type without altering the binary representation.   You can changed the signal between signed and unsigned, and relocate the binary point.<br><br>Hardware notes: In hardware this block costs nothing.<br><br>Example:  Suppose the input is 6 bits wide, signed, with 2 fractional bits, and the output is forced to unsigned with 0 fractional bits.  Then an input of -2.0 (1110.00 in binary 2's complement) becomes an output of 56 (111000 in binary)."
  bus_out : Outport
  wires:
  in1/1 -> reinterpret1/1
  reinterpret1/1 -> bus_out/1

== system snap_adc5g_spec/fft_wideband_real/fft_direct/butterfly0_0/twiddle/bus_mult/repb/bussify ==
  in1 : Inport
  reinterpret1 : xbsIndex_r4/Reinterpret  force_arith_type=on  arith_type=Unsigned  force_bin_pt=on  bin_pt=0  block_type=reinterpret
      settings: infoedit="Changes signal type without altering the binary representation.   You can changed the signal between signed and unsigned, and relocate the binary point.<br><br>Hardware notes: In hardware this block costs nothing.<br><br>Example:  Suppose the input is 6 bits wide, signed, with 2 fractional bits, and the output is forced to unsigned with 0 fractional bits.  Then an input of -2.0 (1110.00 in binary 2's complement) becomes an output of 56 (111000 in binary)."
  bus_out : Outport
  wires:
  in1/1 -> reinterpret1/1
  reinterpret1/1 -> bus_out/1

== system snap_adc5g_spec/fft_wideband_real/fft_direct/butterfly0_0/twiddle/coeff_gen/cosin/add_convert0 ==
  theta : Inport
  misci : Inport  Port=2
  AddSub : xbsIndex_r4/AddSub  mode=Subtraction  use_carryin=off  use_carryout=off  en=off  latency=add_latency  precision=User Defined  arith_type=Unsigned  n_bits=11  bin_pt=0  quantization=Truncate  overflow=Wrap  use_behavioral_HDL=off  hw_selection=Fabric  pipelined=on  dbl_ovrd=off  block_type=addsub
  AddSub5 : xbsIndex_r4/AddSub  mode=Addition  use_carryin=off  use_carryout=off  en=off  latency=0  precision=User Defined  arith_type=Unsigned  n_bits=2  bin_pt=0  quantization=Truncate  overflow=Wrap  use_behavioral_HDL=off  hw_selection=Fabric  pipelined=off  dbl_ovrd=off  block_type=addsub
  Concat : xbsIndex_r4/Concat  num_inputs=2  dbl_ovrd=off  block_type=concat
  Constant4 : xbsIndex_r4/Constant  const=1024  gui_display_data_type=Fixed-point  arith_type=Unsigned  n_bits=11  bin_pt=0  preci_type=Single  exp_width=8  frac_width=24  explicit_period=off  period=1  equ=P=C  opselect=C  inp2=PCIN>>17  opr=+  inp1=P  carry=CIN  dbl_ovrd=off  block_type=constant
  Convert2 : xbsIndex_r4/Convert  gui_display_data_type=Fixed-point  arith_type=Unsigned  n_bits=10  bin_pt=0  float_type=Single  exp_bits=8  fraction_bits=24  quantization=Truncate  overflow=Saturate  en=off  latency=conv_latency  pipeline=on  dbl_ovrd=off  block_type=convert
  Delay1 : xbsIndex_r4/Delay  rst=off  infoeditControl=Selection of Reset will increase slice count due to use of real FFs and instead of SRLs  en=off  latency=mux_latency+add_latency+conv_latency  reg_retiming=on  dbl_ovrd=off  block_type=delay
  Delay13 : xbsIndex_r4/Delay  rst=off  infoeditControl=Selection of Reset will increase slice count due to use of real FFs and instead of SRLs  en=off  latency=add_latency  reg_retiming=off  dbl_ovrd=off  block_type=delay
  Delay14 : xbsIndex_r4/Delay  rst=off  infoeditControl=Selection of Reset will increase slice count due to use of real FFs and instead of SRLs  en=off  latency=add_latency  reg_retiming=off  dbl_ovrd=off  block_type=delay
  Delay2 : xbsIndex_r4/Delay  rst=off  infoeditControl=Selection of Reset will increase slice count due to use of real FFs and instead of SRLs  en=off  latency=add_latency+mux_latency+conv_latency  reg_retiming=on  dbl_ovrd=off  block_type=delay
  Mux : xbsIndex_r4/Mux  inputs=2  en=off  latency=mux_latency  precision=Full  arith_type=Unsigned  n_bits=16  bin_pt=14  quantization=Truncate  overflow=Wrap  dbl_ovrd=off  block_type=mux
  backwards : xbsIndex_r4/Slice  nbits=1  boolean_output=on  mode=Lower Bit Location + Width  bit1=0  base1=MSB of Input  bit0=0  base0=LSB of Input  dbl_ovrd=off  block_type=slice
  direction_offset : xbsIndex_r4/Constant  const=1  gui_display_data_type=Fixed-point  arith_type=Unsigned  n_bits=2  bin_pt=0  preci_type=Single  exp_width=8  frac_width=24  explicit_period=off  period=1  equ=P=C  opselect=C  inp2=PCIN>>17  opr=+  inp1=P  carry=CIN  dbl_ovrd=off  block_type=constant
  fluff : xbsIndex_r4/Concat  num_inputs=2  dbl_ovrd=off  block_type=concat
  invert : xbsIndex_r4/Slice  nbits=1  boolean_output=on  mode=Upper Bit Location + Width  bit1=0  base1=MSB of Input  bit0=0  base0=LSB of Input  dbl_ovrd=off  block_type=slice
  lookup : xbsIndex_r4/Slice  nbits=10  boolean_output=off  mode=Lower Bit Location + Width  bit1=0  base1=MSB of Input  bit0=0  base0=LSB of Input  dbl_ovrd=off  block_type=slice
  new_add : xbsIndex_r4/Slice  nbits=10  boolean_output=off  mode=Lower Bit Location + Width  bit1=0  base1=MSB of Input  bit0=0  base0=LSB of Input  dbl_ovrd=off  block_type=slice
  pad : xbsIndex_r4/Constant  const=0  gui_display_data_type=Fixed-point  arith_type=Unsigned  n_bits=1  bin_pt=0  preci_type=Single  exp_width=8  frac_width=24  explicit_period=off  period=1  equ=P=C  opselect=C  inp2=PCIN>>17  opr=+  inp1=P  carry=CIN  dbl_ovrd=off  block_type=constant
  quadrant : xbsIndex_r4/Slice  nbits=2  boolean_output=off  mode=Upper Bit Location + Width  bit1=0  base1=MSB of Input  bit0=0  base0=LSB of Input  dbl_ovrd=off  block_type=slice
  negate : Outport
  add : Outport  Port=2
  misco : Outport  Port=3
  wires:
  theta/1 -> fluff/2
  pad/1 -> fluff/1
  fluff/1 -> quadrant/1, lookup/1
  direction_offset/1 -> AddSub5/1
  quadrant/1 -> AddSub5/2
  lookup/1 -> Concat/2
  AddSub5/1 -> Concat/1, backwards/1, invert/1
  Concat/1 -> new_add/1
  new_add/1 -> Delay14/1, AddSub/2
  Convert2/1 -> add/1
  backwards/1 -> Delay13/1
  Constant4/1 -> AddSub/1
  Delay13/1 -> Mux/1
  Delay14/1 -> Mux/2
  AddSub/1 -> Mux/3
  Mux/1 -> Convert2/1
  invert/1 -> Delay2/1
  Delay2/1 -> negate/1
  misci/1 -> Delay1/1
  Delay1/1 -> misco/1
